simulink model "Servo_Joint"  (R2026b)
settings: Solver=VariableStepAuto
libraries: fl_lib x5, ee_lib x2, nesl_utility x2, sm_lib x1, sdl_lib x1
settings Model: Creator=controls  LastModifiedBy=controls

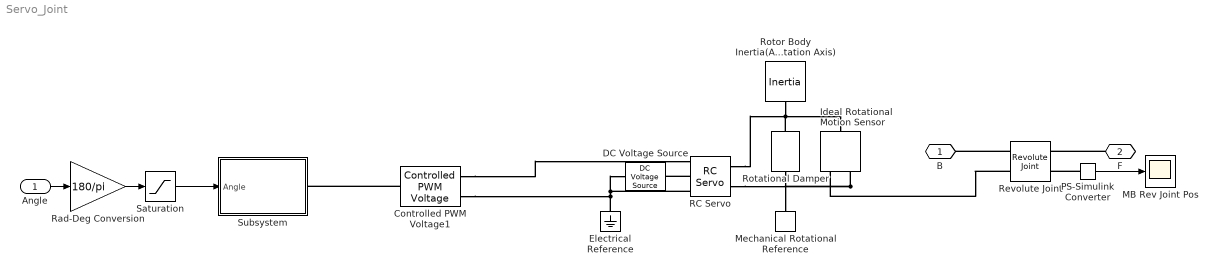
== system Servo_Joint ==
  Angle : Inport
  Controlled PWM Voltage1 : ee_lib/Integrated Circuits/Controlled PWM Voltage  F=50 Hz  TD=0 s  pulse_width_offset=0 s  pulse_min=0 s  pwm_or_av=ee.enum.pwm_or_av.pwm  event_type=ee.enum.ic.event.asynchronous  sample_time=1e-6 s  Vmin=0 V  Vmax=5 V  Vm=5 V  u_min=0  u_max=1
  DC Voltage Source : fl_lib/Electrical/Electrical Sources/DC Voltage Source  v0=12 V
  Electrical Reference : fl_lib/Electrical/Electrical Elements/Electrical Reference
  Ideal Rotational Motion Sensor : fl_lib/Mechanical/Mechanical Sensors/Ideal Rotational Motion Sensor  reference=foundation.enum.MeasurementReference.difference  acceleration_port=false  velocity_port=false  position_port=true  wrap_angle=false  offset=0 rad
  MB Rev Joint Pos : Scope
      settings: ActiveDisplayYMinimum=-0.45947960601207405  ActiveDisplayYMaximum=2.0966132450006238  DataLoggingVariableName=ScopeData5
  Mechanical Rotational Reference : fl_lib/Mechanical/Rotational Elements/Mechanical Rotational Reference
  PS-Simulink Converter : nesl_utility/PS-Simulink Converter  PhysicalDomain=network_engine_domain  SubClassName=ps_output  LeftPortType=input  RightPortType=output  PseudoPeriodic=off  Frequencies=[]  VectorFormat=inherit  Unit=deg  AffineConversion=off
  RC Servo : ee_lib/Electromechanical/Brushed Motors/RC Servo  stall_torque=30.59 cm*kg  time_60=0.1299 s  nominal_voltage=12 V  rotational_range=[0, 180] deg  pulse_width_range=[550, 2330] us  threshold=3 V  R_s=18 kOhm  resolution=0.1 deg  angle_meas_error=0 deg  backdrive_torque=0.5 cm*kg  ratio=212.6  inertia=0.01 cm^2*g  endstop_angles=[-5, 185] deg  endstop_stiffness=1e6 N*m/rad  endstop_damping=0.01 N*m*s/rad  angle_specify=off  angle_priority=High  angle=90 deg  angle_nominal_specify=off  angle_nominal_value=1  angle_nominal_unit=deg  w_specify=off  w_priority=High  w=0 deg/s  w_nominal_specify=off  w_nominal_value=1  w_nominal_unit=deg/s  torque_specify=off  torque_priority=None  torque=0 N*m  torque_nominal_specify=off  torque_nominal_value=1  torque_nominal_unit=N*m  pulse_width_specify=off  pulse_width_priority=Low  pulse_width=1.5 ms  i_specify=off  i_priority=None  i=0 A  i_nominal_specify=off  i_nominal_value=1  i_nominal_unit=A  i_s_specify=off  i_s_priority=None  i_s=0 A  i_s_nominal_specify=off  i_s_nominal_value=1  i_s_nominal_unit=A  motor_torque_specify=off  motor_torque_priority=None  motor_torque=0 N*m  motor_torque_nominal_specify=off  motor_torque_nominal_value=1  motor_torque_nominal_unit=N*m  angle_demand_specify=off  angle_demand_priority=None  angle_demand=90 deg  angle_demand_nominal_specify=off  angle_demand_nominal_value=1  angle_demand_nominal_unit=deg
  Rad-Deg Conversion : Gain  Gain=180/pi
  Revolute Joint : sm_lib/Joints/Revolute Joint  JointMode=Normal  CompositeWrenchDir=FollowerOnBase  CompositeWrenchFrame=BaseFrame  SenseConstraintForce=off  SenseConstraintTorque=off  SenseTotalForce=off  SenseTotalTorque=off  PositionTargetSpecify=off  PositionTargetPriority=High  PositionTargetValue=0  PositionTargetValueUnits=deg  VelocityTargetSpecify=off  VelocityTargetPriority=High  VelocityTargetValue=0  VelocityTargetValueUnits=deg/s  EquilibriumPosition=0  EquilibriumPositionUnits=deg  SpringStiffness=0  SpringStiffnessUnits=N*m/deg  DampingCoefficient=0  DampingCoefficientUnits=N*m/(deg/s)  LowerLimitSpecify=off  LowerLimitBound=-90  LowerLimitBoundUnits=deg  LowerLimitStiffness=1e4  LowerLimitStiffnessUnits=N*m/deg  LowerLimitDamping=10  LowerLimitDampingUnits=N*m/(deg/s)  LowerLimitTransitionRegionWidth=0.1  LowerLimitTransitionRegionWidthUnits=deg  UpperLimitSpecify=off  UpperLimitBound=90  UpperLimitBoundUnits=deg  UpperLimitStiffness=1e4  UpperLimitStiffnessUnits=N*m/deg  UpperLimitDamping=10  UpperLimitDampingUnits=N*m/(deg/s)  UpperLimitTransitionRegionWidth=0.1  UpperLimitTransitionRegionWidthUnits=deg  TorqueActuationMode=ComputedTorque  MotionActuationMode=InputMotion  SensePosition=on  SenseVelocity=off  SenseAcceleration=off  SenseTorqueForce=off  SenseLowerLimitTorqueForce=off  SenseUpperLimitTorqueForce=off
  Rotational Damper : sdl_lib/Couplings & Drives/Springs & Dampers/Rotational Damper  D=0.05 N*m/(deg/s)  thermal_port=simscape.enum.thermaleffects.omit  thermal_mass=50 kJ/K  temperature_specify=off  temperature_priority=High  temperature=300 K  temperature_nominal_specify=off  temperature_nominal_value=1  temperature_nominal_unit=K
  Rotor Body Inertia(About Rotation Axis) : fl_lib/Mechanical/Rotational Elements/Inertia  inertia=0.0039189 kg*m^2  num_ports=foundation.enum.numPorts2.one  w_specify=off  w_priority=High  w=0 rad/s  w_nominal_specify=off  w_nominal_value=1  w_nominal_unit=rad/s  t_specify=off  t_priority=None  t=0 N*m  t_nominal_specify=off  t_nominal_value=1  t_nominal_unit=N*m
  Saturation : Saturate  UpperLimit=30  LowerLimit=-30
  Subsystem : Subsystem
  B : PMIOPort  Side=Left
  F : PMIOPort  Port=2  Side=Right
  wires:
  Angle/1 -> Rad-Deg Conversion/1
  Saturation/1 -> Subsystem/1(Angle)
  PS-Simulink Converter/1 -> MB Rev Joint Pos/1
  Rad-Deg Conversion/1 -> Saturation/1
  connections:
  Rotational Damper/LConn1 -- Rotor Body Inertia(About Rotation Axis)/LConn1 -- RC Servo/RConn1 -- Ideal Rotational Motion Sensor/LConn1
  Controlled PWM Voltage1/RConn2 -- Electrical Reference/LConn1 -- RC Servo/LConn3 -- DC Voltage Source/RConn1
  Ideal Rotational Motion Sensor/RConn1 -- RC Servo/RConn2 -- Rotational Damper/RConn1 -- Mechanical Rotational Reference/LConn1
  Controlled PWM Voltage1/RConn1 -- RC Servo/LConn1
  F/RConn1 -- Revolute Joint/RConn1
  Revolute Joint/LConn1 -- B/RConn1
  RC Servo/LConn2 -- DC Voltage Source/LConn1
  PS-Simulink Converter/LConn1 -- Revolute Joint/RConn2
  Revolute Joint/LConn2 -- Ideal Rotational Motion Sensor/RConn2
  Controlled PWM Voltage1/LConn1 -- Subsystem/RConn1

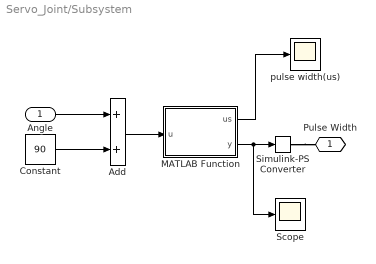
== system Servo_Joint/Subsystem ==
  Angle : Inport
  Add : Sum
  Constant : Constant  Value=90
  MATLAB Function : MATLAB Function  TreatAsAtomicUnit=on
  Scope : Scope
      settings: ActiveDisplayYMinimum=0.072283897596501792  ActiveDisplayYMaximum=0.072285872557738176  DataLoggingVariableName=ScopeData8
  Simulink-PS Converter : nesl_utility/Simulink-PS Converter  PhysicalDomain=network_engine_domain  SubClassName=ps_input  LeftPortType=input  RightPortType=output  PseudoPeriodic=off  Frequencies=[]  NoiseDistribution=none  NoiseParameters=[]  Unit=1  AffineConversion=off  FilteringAndDerivatives=provide  SimscapeFilterOrder=1  InputFilterTimeConstant=0.001  UdotUserProvided=0
  pulse width(us) : Scope
      settings: ActiveDisplayYMinimum=1443.3126434212586  ActiveDisplayYMaximum=1443.3281354688727  DataLoggingVariableName=ScopeData4
  Pulse Width : PMIOPort  Side=Right
  wires:
  MATLAB Function/1(us) -> pulse width(us)/1
  Add/1 -> MATLAB Function/1(u)
  Constant/1 -> Add/2
  MATLAB Function/2(y) -> Simulink-PS Converter/1, Scope/1
  Angle/1 -> Add/1
  connections:
  Simulink-PS Converter/RConn1 -- Pulse Width/RConn1

== matlab function Servo_Joint/Subsystem/MATLAB Function ==
  data: us output; u input; y output
function [us, y]= fcn(u)
freq = 50
T = 1000000/(freq)

aup = 180
alow = 0

mup = 2330
mlow = 550

us = (mup-mlow)*(u-alow)/(aup-alow) + mlow 

y = us / T
